simulink subsystem "State_Estimator_Model"  (R2025b)
settings: Solver=VariableStepAuto  StartTime=0.0  StopTime=10.0  RelTol=1e-3
undefined symbols (not defined in the file): dspblkCoreblockFVToolHelper, dt, gcbh, P_init, x_init
settings Model: Creator=Admin  LastModifiedBy=Admin

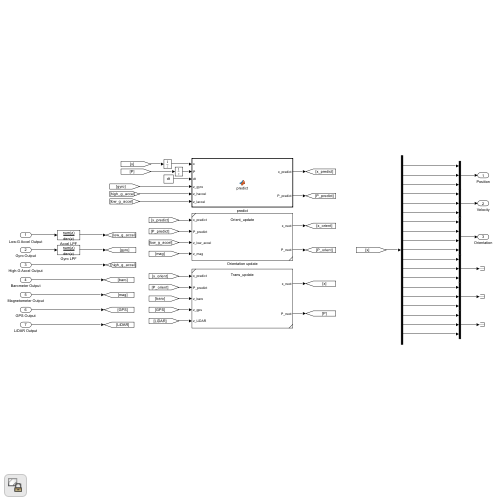
[thumbnail: Simulink's stored preview of the top-level diagram]
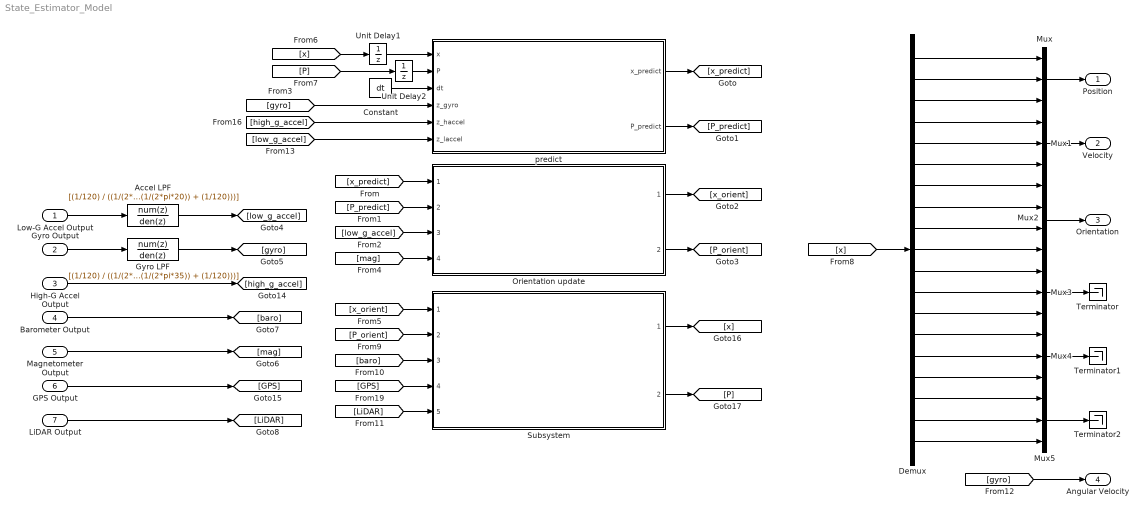
== system State_Estimator_Model ==
  Low-G Accel Output : Inport
  Gyro Output : Inport  Port=2
  High-G Accel Output : Inport  Port=3
  Barometer Output : Inport  Port=4
  Magnetometer Output : Inport  Port=5
  GPS Output : Inport  Port=6
  LiDAR Output : Inport  Port=7
  Accel LPF : DiscreteFilter  LoadFcn=dspblkCoreblockFVToolHelper(gcbh,'load');  Numerator=[(1/120) / ((1/(2*pi*20)) + (1/120))]  Denominator=[1, -1 + ((1/120) / ((1/(2*pi*20)) + (1/120)))]
      settings: CopyFcn=dspblkCoreblockFVToolHelper(gcbh,'copy');  DeleteFcn=dspblkCoreblockFVToolHelper(gcbh,'close');  ModelCloseFcn=dspblkCoreblockFVToolHelper(gcbh,'close');  PreSaveFcn=dspblkCoreblockFVToolHelper(gcbh,'presave');  PostSaveFcn=dspblkCoreblockFVToolHelper(gcbh,'postsave');  CloseFcn=dspblkCoreblockFVToolHelper(gcbh,'close');
  Constant : Constant  Value=dt
  Demux : Demux  Outputs=19
  Gyro LPF : DiscreteFilter  LoadFcn=dspblkCoreblockFVToolHelper(gcbh,'load');  Numerator=[(1/120) / ((1/(2*pi*35)) + (1/120))]  Denominator=[1, -1 + ((1/120) / ((1/(2*pi*35)) + (1/120)))]
      settings: CopyFcn=dspblkCoreblockFVToolHelper(gcbh,'copy');  DeleteFcn=dspblkCoreblockFVToolHelper(gcbh,'close');  ModelCloseFcn=dspblkCoreblockFVToolHelper(gcbh,'close');  PreSaveFcn=dspblkCoreblockFVToolHelper(gcbh,'presave');  PostSaveFcn=dspblkCoreblockFVToolHelper(gcbh,'postsave');  CloseFcn=dspblkCoreblockFVToolHelper(gcbh,'close');
  Mux{,1,3..5} (5 alike) : Mux  Inputs=3
  Mux2 : Mux
  Orientation update : Subsystem  ReferencedSubsystem=Orient_update
  Subsystem : Subsystem  ReferencedSubsystem=Trans_update
  Terminator : Terminator
  Terminator1 : Terminator
  Terminator2 : Terminator
  Unit Delay1 : UnitDelay  InitialCondition=x_init  SampleTime=dt  HasFrameUpgradeWarning=on
  Unit Delay2 : UnitDelay  InitialCondition=P_init  SampleTime=dt  HasFrameUpgradeWarning=on
  predict : MATLAB Function  TreatAsAtomicUnit=on
  Position : Outport
  Velocity : Outport  Port=2
  Orientation : Outport  Port=3
  Angular Velocity : Outport  Port=4
  wires:
  Unit Delay2/1 -> predict/2(P)
  Unit Delay1/1 -> predict/1(x)
  Constant/1 -> predict/3(dt)
  [x] -> Unit Delay1/1
  [P] -> Unit Delay2/1
  [P_predict] -> Orientation update/2
  [x_predict] -> Orientation update/1
  Low-G Accel Output/1 -> Accel LPF/1
  Magnetometer Output/1 -> [mag]
  [mag] -> Orientation update/4
  Barometer Output/1 -> [baro]
  High-G Accel Output/1 -> [high_g_accel]
  [x] -> Demux/1
  GPS Output/1 -> [GPS]
  [x_orient] -> Subsystem/1
  [P_orient] -> Subsystem/2
  [baro] -> Subsystem/3
  [GPS] -> Subsystem/4
  Orientation update/1 -> [x_orient]
  Orientation update/2 -> [P_orient]
  [low_g_accel] -> Orientation update/3
  [high_g_accel] -> predict/5(z_haccel)
  [gyro] -> predict/4(z_gyro)
  [low_g_accel] -> predict/6(z_laccel)
  predict/2(P_predict) -> [P_predict]
  predict/1(x_predict) -> [x_predict]
  Demux/1 -> Mux/1
  Demux/2 -> Mux/2
  Demux/3 -> Mux/3
  Mux/1 -> Position/1
  Demux/7 -> Mux2/1
  Demux/9 -> Mux2/3
  Demux/8 -> Mux2/2
  Demux/10 -> Mux2/4
  Mux2/1 -> Orientation/1
  Mux1/1 -> Velocity/1
  Demux/5 -> Mux1/2
  Demux/4 -> Mux1/1
  Demux/6 -> Mux1/3
  Mux3/1 -> Terminator/1
  Demux/12 -> Mux3/2
  Demux/11 -> Mux3/1
  Demux/13 -> Mux3/3
  Mux4/1 -> Terminator1/1
  Demux/15 -> Mux4/2
  Demux/14 -> Mux4/1
  Demux/16 -> Mux4/3
  Mux5/1 -> Terminator2/1
  Demux/18 -> Mux5/2
  Demux/17 -> Mux5/1
  Demux/19 -> Mux5/3
  Subsystem/1 -> [x]
  Subsystem/2 -> [P]
  LiDAR Output/1 -> [LiDAR]
  [LiDAR] -> Subsystem/5
  Gyro Output/1 -> Gyro LPF/1
  Gyro LPF/1 -> [gyro]
  Accel LPF/1 -> [low_g_accel]
  [gyro] -> Angular Velocity/1

== matlab function State_Estimator_Model/predict ==
  data: x input; x_predict output; P input; P_predict output; dt input; z_gyro input; z_haccel input; z_laccel input
function [x_predict, P_predict] = predict(x, P, dt, z_gyro, z_haccel, z_laccel)
%PREDICT  EKF predict step — IMU used as control input (u vector)
%
%  State:  x = [p(3); v(3); q(4); bg(3); ba_high(3); ba_low(3)]  (19x1)
%  Inputs: z_gyro   — raw gyro measurement         [rad/s]
%          z_haccel — raw high-G accel measurement  [m/s^2]
%          z_laccel — raw low-G  accel measurement  [m/s^2]

I3    = eye(3);
g_vec = [0; 0; 9.81];   % NED: gravity along +Z. Flip sign for ENU.

%% ── Extract states ───────────────────────────────────────────────────────────
%   p  : 1:3    v  : 4:6    q  : 7:10
%   bg : 11:13  ba_high : 14:16  ba_low : 17:19
p       = x(1:3);
v       = x(4:6);
q       = x(7:10);   q = q / norm(q);
bg      = x(11:13);
ba_high = x(14:16);
ba_low  = x(17:19);

q0=q(1); q1=q(2); q2=q(3); q3=q(4);

%% ── R body→NED: built from body2ned on basis vectors ────────────────────────
%  Only needed for the F Jacobian bias-coupling blocks (∂p,∂v / ∂ba).
%  All vector rotations below use body2ned / ned2body directly.
R = [body2ned([1;0;0], q), ...
     body2ned([0;1;0], q), ...
     body2ned([0;0;1], q)];   % 3×3

%% ── Hard accel switch at 7g ──────────────────────────────────────────────────
THRESHOLD_G = 7 * 9.81;   % [m/s^2]
use_high_g  = norm(z_haccel) <= THRESHOLD_G;

if use_high_g
    a_corr = z_haccel - ba_high;
else
    a_corr = z_laccel - ba_low;
end

%% ── Correct gyro + rotate accel to NED world frame ──────────────────────────
w_corr  = z_gyro - bg;
a_world = body2ned(a_corr, q) + g_vec;   % specific force → NED, remove gravity

%% ── Attitude propagation (closed-form matrix exponential) ───────────────────
wx=w_corr(1); wy=w_corr(2); wz=w_corr(3);
Omega = [  0   -wx  -wy  -wz;
           wx   0    wz  -wy;
           wy  -wz   0    wx;
           wz   wy  -wx   0  ];

w_norm = norm(w_corr);
if w_norm > 1e-9
    F_qq = cos(0.5*w_norm*dt)*eye(4) + (sin(0.5*w_norm*dt)/w_norm)*0.5*Omega;
else
    F_qq = eye(4) + 0.5*dt*Omega;
end

% E_q: maps body-frame angular velocity → quaternion derivative
E_q = [-q1 -q2 -q3;
        q0 -q3  q2;
        q3  q0 -q1;
       -q2  q1  q0];

F_qw  =  0.5*dt * E_q;   % ∂q_new/∂w_corr  [4×3]
F_qbg = -F_qw;           % ∂q_new/∂bg      [4×3]

%% ── Jacobian ∂(body2ned(a_corr,q))/∂q  [3×4] ───────────────────────────────
vx=a_corr(1); vy=a_corr(2); vz=a_corr(3);
dRa_dq = 2*...
  [ q0*vx - q3*vy + q2*vz,   q1*vx + q2*vy + q3*vz,  -q2*vx + q1*vy + q0*vz,  -q3*vx - q0*vy + q1*vz;
    q3*vx + q0*vy - q1*vz,   q2*vx - q1*vy - q0*vz,   q1*vx + q2*vy + q3*vz,  -q0*vx - q3*vy + q2*vz;
   -q2*vx + q1*vy + q0*vz,   q3*vx + q0*vy - q1*vz,  -q0*vx + q3*vy - q2*vz,   q1*vx + q2*vy + q3*vz];

%% ── State transition Jacobian F [19×19] ──────────────────────────────────────
F = eye(19);

% ── Kinematic chain ──
F(1:3,  4:6)  =  dt * I3;               % ∂p_new/∂v

% ── Cross-coupling: [p,v] ↔ quaternion (through body2ned(a_corr,q)) ──
F(1:3,  7:10) =  0.5*dt^2 * dRa_dq;    % ∂p_new/∂q
F(4:6,  7:10) =       dt   * dRa_dq;   % ∂v_new/∂q

% ── Cross-coupling: [p,v] ↔ active accel bias (through -R) ──
if use_high_g
    F(1:3,  14:16) = -0.5*dt^2 * R;    % ∂p_new/∂ba_high
    F(4:6,  14:16) =      -dt   * R;   % ∂v_new/∂ba_high
else
    F(1:3,  17:19) = -0.5*dt^2 * R;    % ∂p_new/∂ba_low
    F(4:6,  17:19) =      -dt   * R;   % ∂v_new/∂ba_low
end

% ── Quaternion block ──
F(7:10,  7:10) = F_qq;                  % ∂q_new/∂q_old
F(7:10, 11:13) = F_qbg;                % ∂q_new/∂bg

% ── Biases: random walk — I3 blocks already set by eye(19) ──

%% ── Process noise Q [19×19] ──────────────────────────────────────────────────
sigma_w_meas  = diag([0.05, 0.03, 0.03]);   % gyro  noise  [rad/s/√Hz]  — from datasheet ARW
sigma_bg      = diag([5e-5, 5e-5, 5e-5]);  % gyro  bias instability     [rad/s/√s]
sigma_ba_high = 0.002;   % high-G bias instability    [m/s^2/√s]
sigma_ba_low  = diag([5e-4, 5e-4, 5e-4]);   % low-G  bias instability    [m/s^2/√s]

if use_high_g
    sigma_a_meas = 0.1 * I3;  % high-G noise [m/s^2/√Hz]  — from datasheet VRW
else
    sigma_a_meas = diag([0.008, 0.006, 0.004]); % low-G  noise [m/s^2/√Hz]  — tighter at low-G
end

% Accel noise propagated into [p; v] via kinematic input matrix
G_trans = [0.5*dt^2 * I3;
                 dt  * I3];                                     % 6×3
Q_trans = G_trans * (sigma_a_meas.^2) * G_trans';          % 6×6

% Gyro noise propagated into q (no w state)
G_att = 0.5*dt * E_q;                                          % 4×3
Q_att = G_att * (sigma_w_meas^2) * G_att';                % 4×4

Q_bg      = (sigma_bg^2      * dt);
Q_ba_high = (sigma_ba_high^2 * dt) * I3;
Q_ba_low  = (sigma_ba_low^2  * dt);

Q = blkdiag(Q_trans, Q_att, Q_bg, Q_ba_high, Q_ba_low);        % 19×19

%% ── Predict state ────────────────────────────────────────────────────────────
x_predict = zeros(19,1);

x_predict(1:3)   = p + v*dt + 0.5*a_world*dt^2;
x_predict(4:6)   = v + a_world*dt;
x_predict(7:10)  = F_qq * q;
x_predict(7:10)  = x_predict(7:10) / norm(x_predict(7:10));
x_predict(11:13) = bg;
x_predict(14:16) = ba_high;
x_predict(17:19) = ba_low;

%% ── Predict covariance ───────────────────────────────────────────────────────
P_predict = F * P * F' + Q;
P_predict = 0.5 * (P_predict + P_predict');

end
